simulink library "focLib"  (R2023a)
settings: Solver=VariableStepAuto  StartTime=0.0  StopTime=10.0  RelTol=1e-3
undefined symbols (not defined in the file): availableSpeedModes, ctrl_limits, Down, focp_tune_cur_Ki, focp_tune_cur_Kp, focp_tune_iq_max, focp_tune_iq_min, focp_tune_spd_Ki, focp_tune_spd_Kp, focp_tune_udc_max, GPTRIP1SEL, inverter_DRV8300, PI_params, pmsm_ECI6360, PU_System, target_f2838, Ts, Ts_motor, Ts_simulink, Ts_speed, TZ1, Up
libraries: simulink x31, c2802xlib x12, idelinklib_common x8, mcbcontrolslib x8, c280xlib x7, mcbpositiondecoderlib x7, slpidlib x5, c2837xDlib x2, c2838xlib x1, autolibpmsminterior x1, mcbplantlib x1, autolibpmsmexterior x1
(part 1 of 3)
Description:
  | FOC-Framework Komponentenbibliothek. Aus impmodel erzeugt durch foc_build_library am 2026-11-03 11:16
settings Model: Creator=Student  LastModifiedBy=Student

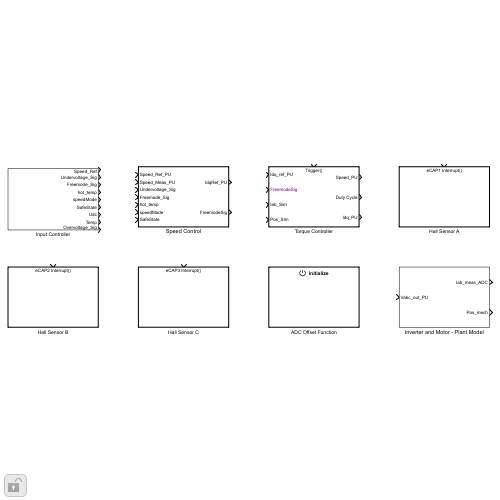
[thumbnail: Simulink's stored preview of the top-level diagram]
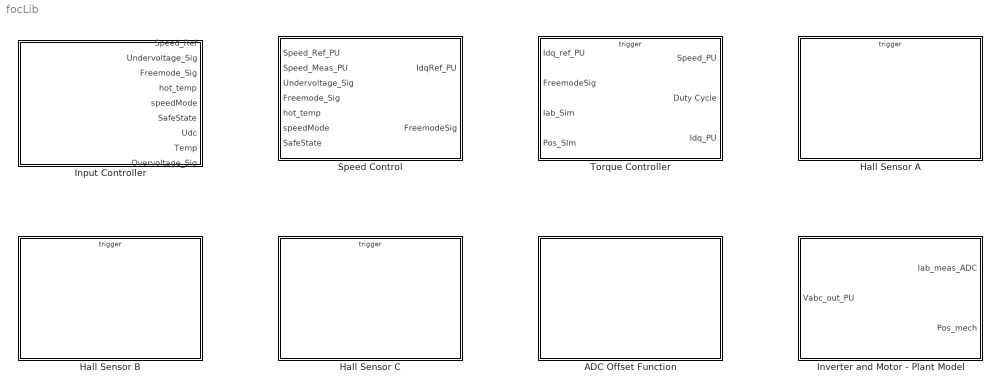
== system focLib ==
  ADC Offset Function : Subsystem  TreatAsAtomicUnit=on
  Hall Sensor A : Subsystem
  Hall Sensor B : Subsystem
  Hall Sensor C : Subsystem
  Input Controller : Subsystem
  Inverter and Motor - Plant Model : Subsystem
  Speed Control : Subsystem  TreatAsAtomicUnit=on  SystemSampleTime=Ts_speed
  Torque Controller : Subsystem

== system focLib/ADC Offset Function ==
  "Calculate ADC Offset " : Subsystem  Priority=1001  TreatAsAtomicUnit=on
  Constant : Constant  Value=inverter_DRV8300.ADCOffsetCalibEnable
  Default ADC Offset : Subsystem  Priority=1001  TreatAsAtomicUnit=on
  Event Listener : EventListener  DisableCoverage=on  EventName=reset
  NOT : Logic  Operator=NOT  IconShape=distinctive  AllPortsSameDT=off  OutDataTypeStr=boolean
  wires:
  NOT/1 -> Default ADC Offset/Enable
  Constant/1 -> "Calculate ADC Offset "/Enable, NOT/1

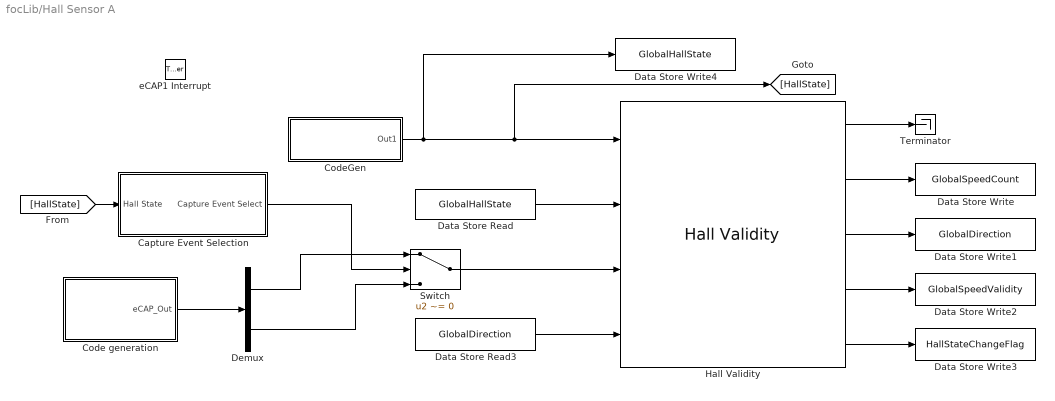
== system focLib/Hall Sensor A ==
  eCAP1 Interrupt : TriggerPort  TriggerType=function-call  VariantControl=(inherit)  PortDimensions=1
  Capture Event Selection : Subsystem
  Code generation : Subsystem
  CodeGen : Subsystem
  Data Store Read : DataStoreRead  DataStoreName=GlobalHallState  IndexOptions=Index vector (dialog)  Indices=1  OutputSizes=1
  Data Store Read3 : DataStoreRead  DataStoreName=GlobalDirection  IndexOptions=Index vector (dialog)  Indices=1  OutputSizes=1
  Data Store Write : DataStoreWrite  DataStoreName=GlobalSpeedCount  IndexOptions=Index vector (dialog)  Indices=1  OutputSizes=1
  Data Store Write1 : DataStoreWrite  DataStoreName=GlobalDirection  IndexOptions=Index vector (dialog)  Indices=1  OutputSizes=1
  Data Store Write2 : DataStoreWrite  DataStoreName=GlobalSpeedValidity  IndexOptions=Index vector (dialog)  Indices=1  OutputSizes=1
  Data Store Write3 : DataStoreWrite  DataStoreName=HallStateChangeFlag  IndexOptions=Index vector (dialog)  Indices=1  OutputSizes=1
  Data Store Write4 : DataStoreWrite  DataStoreName=GlobalHallState  IndexOptions=Index vector (dialog)  Indices=1  OutputSizes=1
  Demux : Demux  Outputs=2
  Hall Validity : mcbpositiondecoderlib/Hall Validity  hallSequence=ABC  sequence=[5,4,6,2,3,1]  CounterSize=32 bits
      settings: LibrarySourceBlock=mcblib/Sensor Decoders/Hall Validity
  Switch : Switch  Criteria=u2 ~= 0  SaturateOnIntegerOverflow=off  InputSameDT=off
  Terminator : Terminator
  wires:
  Demux/2 -> Switch/3
  Demux/1 -> Switch/1
  Data Store Read/1 -> Hall Validity/2
  Code generation/1(eCAP_Out) -> Demux/1
  Capture Event Selection/1(Capture Event Select) -> Switch/2
  Switch/1 -> Hall Validity/3
  [HallState] -> Capture Event Selection/1(Hall State)
  Hall Validity/3 -> Data Store Write1/1
  Hall Validity/2 -> Data Store Write/1
  CodeGen/1(Out1) -> Data Store Write4/1, [HallState], Hall Validity/1
  Data Store Read3/1 -> Hall Validity/4
  Hall Validity/5 -> Data Store Write3/1
  Hall Validity/1 -> Terminator/1
  Hall Validity/4 -> Data Store Write2/1

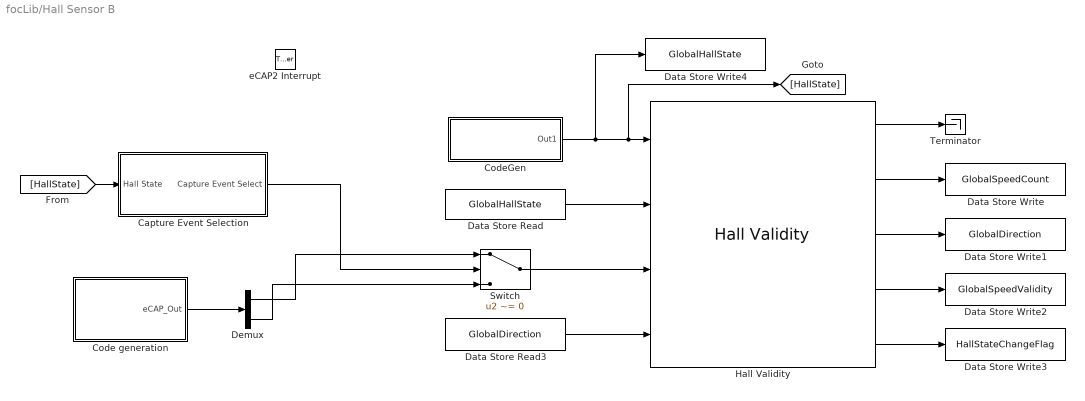
== system focLib/Hall Sensor B ==
  eCAP2 Interrupt : TriggerPort  TriggerType=function-call  VariantControl=(inherit)  PortDimensions=1
  Capture Event Selection : Subsystem
  Code generation : Subsystem
  CodeGen : Subsystem
  Data Store Read : DataStoreRead  DataStoreName=GlobalHallState  IndexOptions=Index vector (dialog)  Indices=1  OutputSizes=1
  Data Store Read3 : DataStoreRead  DataStoreName=GlobalDirection  IndexOptions=Index vector (dialog)  Indices=1  OutputSizes=1
  Data Store Write : DataStoreWrite  DataStoreName=GlobalSpeedCount  IndexOptions=Index vector (dialog)  Indices=1  OutputSizes=1
  Data Store Write1 : DataStoreWrite  DataStoreName=GlobalDirection  IndexOptions=Index vector (dialog)  Indices=1  OutputSizes=1
  Data Store Write2 : DataStoreWrite  DataStoreName=GlobalSpeedValidity  IndexOptions=Index vector (dialog)  Indices=1  OutputSizes=1
  Data Store Write3 : DataStoreWrite  DataStoreName=HallStateChangeFlag  IndexOptions=Index vector (dialog)  Indices=1  OutputSizes=1
  Data Store Write4 : DataStoreWrite  DataStoreName=GlobalHallState  IndexOptions=Index vector (dialog)  Indices=1  OutputSizes=1
  Demux : Demux  Outputs=2
  Hall Validity : mcbpositiondecoderlib/Hall Validity  hallSequence=ABC  sequence=[5,4,6,2,3,1]  CounterSize=32 bits
      settings: LibrarySourceBlock=mcblib/Sensor Decoders/Hall Validity
  Switch : Switch  Criteria=u2 ~= 0  SaturateOnIntegerOverflow=off  InputSameDT=off
  Terminator : Terminator
  wires:
  Data Store Read/1 -> Hall Validity/2
  Switch/1 -> Hall Validity/3
  Demux/2 -> Switch/3
  Demux/1 -> Switch/1
  Code generation/1(eCAP_Out) -> Demux/1
  [HallState] -> Capture Event Selection/1(Hall State)
  Capture Event Selection/1(Capture Event Select) -> Switch/2
  Hall Validity/4 -> Data Store Write2/1
  Hall Validity/1 -> Terminator/1
  Hall Validity/5 -> Data Store Write3/1
  Data Store Read3/1 -> Hall Validity/4
  CodeGen/1(Out1) -> Data Store Write4/1, Hall Validity/1, [HallState]
  Hall Validity/2 -> Data Store Write/1
  Hall Validity/3 -> Data Store Write1/1

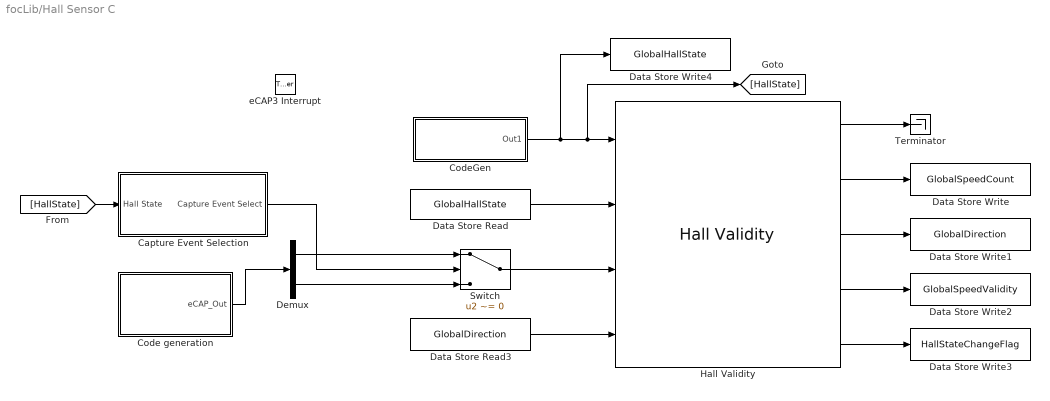
== system focLib/Hall Sensor C ==
  eCAP3 Interrupt : TriggerPort  TriggerType=function-call  VariantControl=(inherit)  PortDimensions=1
  Capture Event Selection : Subsystem
  Code generation : Subsystem
  CodeGen : Subsystem
  Data Store Read : DataStoreRead  DataStoreName=GlobalHallState  IndexOptions=Index vector (dialog)  Indices=1  OutputSizes=1
  Data Store Read3 : DataStoreRead  DataStoreName=GlobalDirection  IndexOptions=Index vector (dialog)  Indices=1  OutputSizes=1
  Data Store Write : DataStoreWrite  DataStoreName=GlobalSpeedCount  IndexOptions=Index vector (dialog)  Indices=1  OutputSizes=1
  Data Store Write1 : DataStoreWrite  DataStoreName=GlobalDirection  IndexOptions=Index vector (dialog)  Indices=1  OutputSizes=1
  Data Store Write2 : DataStoreWrite  DataStoreName=GlobalSpeedValidity  IndexOptions=Index vector (dialog)  Indices=1  OutputSizes=1
  Data Store Write3 : DataStoreWrite  DataStoreName=HallStateChangeFlag  IndexOptions=Index vector (dialog)  Indices=1  OutputSizes=1
  Data Store Write4 : DataStoreWrite  DataStoreName=GlobalHallState  IndexOptions=Index vector (dialog)  Indices=1  OutputSizes=1
  Demux : Demux  Outputs=2
  Hall Validity : mcbpositiondecoderlib/Hall Validity  hallSequence=ABC  sequence=[5,4,6,2,3,1]  CounterSize=32 bits
      settings: LibrarySourceBlock=mcblib/Sensor Decoders/Hall Validity
  Switch : Switch  Criteria=u2 ~= 0  SaturateOnIntegerOverflow=off  InputSameDT=off
  Terminator : Terminator
  wires:
  Data Store Read/1 -> Hall Validity/2
  Capture Event Selection/1(Capture Event Select) -> Switch/2
  Demux/2 -> Switch/3
  Demux/1 -> Switch/1
  Code generation/1(eCAP_Out) -> Demux/1
  Switch/1 -> Hall Validity/3
  [HallState] -> Capture Event Selection/1(Hall State)
  Hall Validity/3 -> Data Store Write1/1
  Hall Validity/2 -> Data Store Write/1
  CodeGen/1(Out1) -> Hall Validity/1, [HallState], Data Store Write4/1
  Data Store Read3/1 -> Hall Validity/4
  Hall Validity/5 -> Data Store Write3/1
  Hall Validity/1 -> Terminator/1
  Hall Validity/4 -> Data Store Write2/1

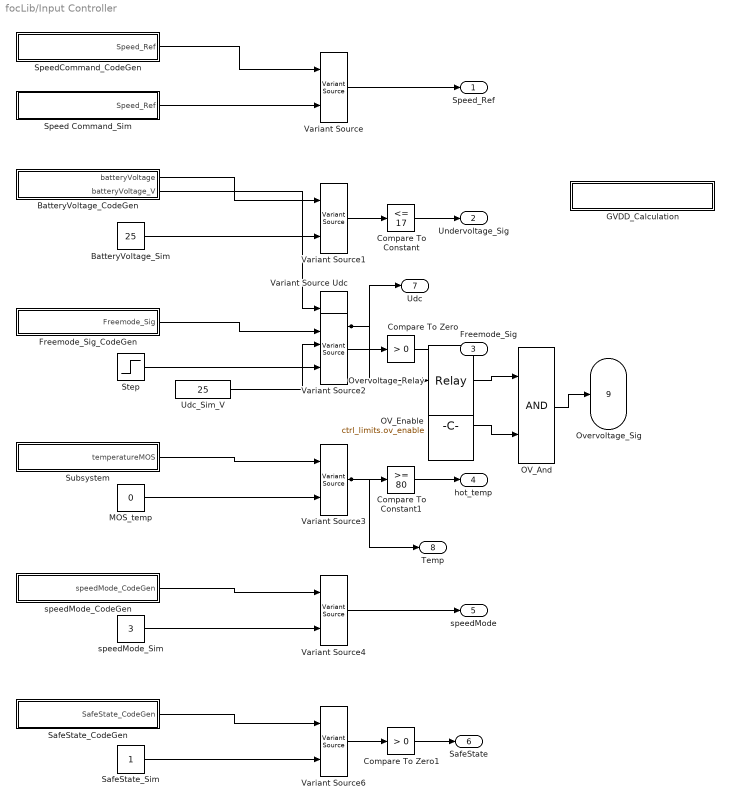
== system focLib/Input Controller ==
  BatteryVoltage_CodeGen : Subsystem
  BatteryVoltage_Sim : Constant  Value=25  OutDataTypeStr=uint16  SampleTime=0.2
  Compare To Constant : simulink/Logic and Bit Operations/Compare To Constant  relop=<=  const=17  OutDataTypeStr=boolean
  Compare To Constant1 : simulink/Logic and Bit Operations/Compare To Constant  relop=>=  const=80  OutDataTypeStr=boolean
  Compare To Zero : simulink/Logic and Bit Operations/Compare To Zero  relop=>  OutDataTypeStr=boolean
  Compare To Zero1 : simulink/Logic and Bit Operations/Compare To Zero  relop=>  OutDataTypeStr=boolean
  Freemode_Sig_CodeGen : Subsystem
  GVDD_Calculation : Subsystem
  MOS_temp : Constant  Value=0  OutDataTypeStr=uint16  SampleTime=0.2
  OV_And : Logic  AllPortsSameDT=off  OutDataTypeStr=boolean
  OV_Enable : Constant  Value=ctrl_limits.ov_enable  OutDataTypeStr=boolean
  Overvoltage_Relay : Relay  OnSwitchValue=focp_tune_udc_max  OffSwitchValue=focp_tune_udc_max - ctrl_limits.Udc_hyst  OutDataTypeStr=boolean
  SafeState_CodeGen : Subsystem
  SafeState_Sim : Constant  OutDataTypeStr=uint8  SampleTime=0.2
  Speed Command_Sim : Subsystem
  SpeedCommand_CodeGen : Subsystem
  Step : Step  Time=10  After=0  SampleTime=0.2
  Subsystem : Subsystem
  Udc_Sim_V : Constant  Value=25  OutDataTypeStr=single
  Variant Source{,1..4,6} (6 alike) : VariantSource  VariantControlMode=sim codegen switching
  Variant Source Udc : VariantSource  VariantControlMode=sim codegen switching
  speedMode_CodeGen : Subsystem
  speedMode_Sim : Constant  Value=3  OutDataTypeStr=uint16  SampleTime=0.2
  Speed_Ref : Outport
  Undervoltage_Sig : Outport  Port=2
  Freemode_Sig : Outport  Port=3
  hot_temp : Outport  Port=4
  speedMode : Outport  Port=5
  SafeState : Outport  Port=6
  Udc : Outport  Port=7
  Temp : Outport  Port=8
  Overvoltage_Sig : Outport  Port=9
  wires:
  Compare To Zero1/1 -> SafeState/1
  SafeState_CodeGen/1(SafeState_CodeGen) -> Variant Source6/1
  SafeState_Sim/1 -> Variant Source6/2
  Variant Source6/1 -> Compare To Zero1/1
  Compare To Zero/1 -> Freemode_Sig/1
  speedMode_CodeGen/1(speedMode_CodeGen) -> Variant Source4/1
  speedMode_Sim/1 -> Variant Source4/2
  Variant Source4/1 -> speedMode/1
  Compare To Constant1/1 -> hot_temp/1
  Variant Source3/1 -> Compare To Constant1/1, Temp/1
  MOS_temp/1 -> Variant Source3/2
  Subsystem/1(temperatureMOS) -> Variant Source3/1
  Freemode_Sig_CodeGen/1(Freemode_Sig) -> Variant Source2/1
  Step/1 -> Variant Source2/2
  Variant Source2/1 -> Compare To Zero/1
  Compare To Constant/1 -> Undervoltage_Sig/1
  BatteryVoltage_Sim/1 -> Variant Source1/2
  BatteryVoltage_CodeGen/1(batteryVoltage) -> Variant Source1/1
  Variant Source1/1 -> Compare To Constant/1
  Speed Command_Sim/1(Speed_Ref) -> Variant Source/2
  SpeedCommand_CodeGen/1(Speed_Ref) -> Variant Source/1
  Variant Source/1 -> Speed_Ref/1
  BatteryVoltage_CodeGen/2(batteryVoltage_V) -> Variant Source Udc/1
  Udc_Sim_V/1 -> Variant Source Udc/2
  Variant Source Udc/1 -> Udc/1, Overvoltage_Relay/1
  Overvoltage_Relay/1 -> OV_And/1
  OV_Enable/1 -> OV_And/2
  OV_And/1 -> Overvoltage_Sig/1

== system focLib/Inverter and Motor - Plant Model ==
  Vabc_out_PU : Inport
  Codegeneration : Subsystem
  Simulation : Subsystem
  Variant Sink : VariantSink  VariantControlMode=sim codegen switching
  Variant Source : VariantSource  VariantControlMode=sim codegen switching
  Variant Source1 : VariantSource  VariantControlMode=sim codegen switching
  Iab_meas_ADC : Outport  VectorParamsAs1DForOutWhenUnconnected=off
  Pos_mech : Outport  Port=2  VectorParamsAs1DForOutWhenUnconnected=off
  wires:
  Vabc_out_PU/1 -> Variant Sink/1
  Simulation/2(Pos_fb_Sim) -> Variant Source1/2
  Variant Sink/2 -> Simulation/1(Duty_Cycles)
  Simulation/1(Iab_fb_Sim) -> Variant Source/2
  Variant Source/1 -> Iab_meas_ADC/1
  Variant Sink/1 -> Codegeneration/1(Duty_Cycles)
  Variant Source1/1 -> Pos_mech/1
  Codegeneration/1(Iab_fb_Sim) -> Variant Source/1
  Codegeneration/2(Pos_fb_Sim) -> Variant Source1/1

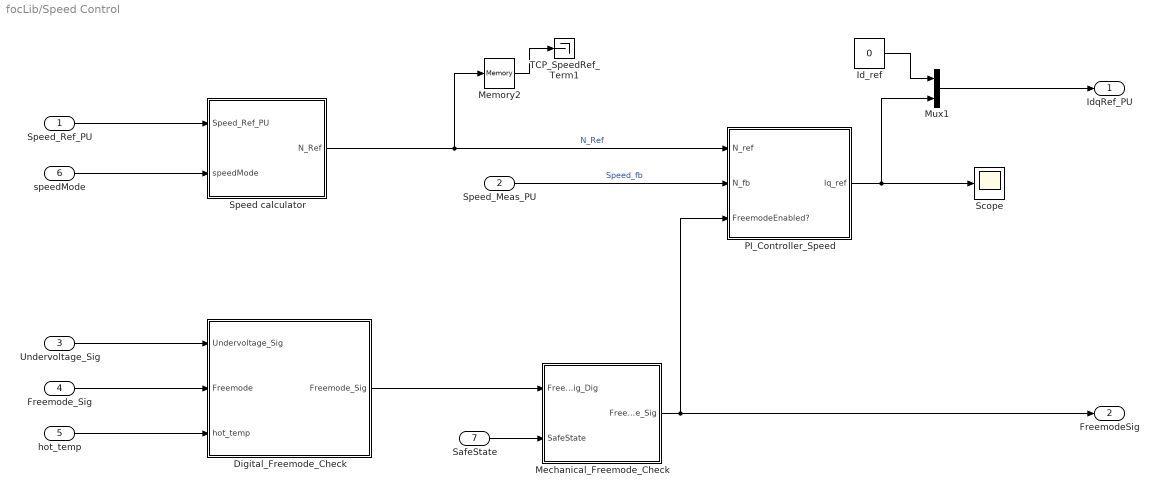
== system focLib/Speed Control ==
  Speed_Ref_PU : Inport
  Speed_Meas_PU : Inport  Port=2
  Undervoltage_Sig : Inport  Port=3
  Freemode_Sig : Inport  Port=4
  hot_temp : Inport  Port=5
  speedMode : Inport  Port=6
  SafeState : Inport  Port=7
  Digital_Freemode_Check : Subsystem  TreatAsAtomicUnit=on
  Id_ref : Constant  Value=0  OutDataTypeStr=fixdt(1,32,17)  SampleTime=Ts_speed
  Mechanical_Freemode_Check : Subsystem
  Memory2 : Memory  InheritSampleTime=on
  Mux1 : Mux  Inputs=2
  PI_Controller_Speed : Subsystem  TreatAsAtomicUnit=on  SystemSampleTime=Ts_speed
  Scope : Scope
  Speed calculator : Subsystem
  TCP_SpeedRef_Term1 : Terminator
  IdqRef_PU : Outport  VectorParamsAs1DForOutWhenUnconnected=off
  FreemodeSig : Outport  Port=2  VectorParamsAs1DForOutWhenUnconnected=off
  wires:
  Mechanical_Freemode_Check/1(Freemode_Sig) -> FreemodeSig/1, PI_Controller_Speed/3("  FreemodeEnabled?")
  Digital_Freemode_Check/1("Freemode_Sig  ") -> Mechanical_Freemode_Check/1(Freemode_Sig_Dig)
  PI_Controller_Speed/1(Iq_ref) -> Mux1/2, Scope/1
  SafeState/1 -> Mechanical_Freemode_Check/2(SafeState)
  Speed_Ref_PU/1 -> Speed calculator/1(Speed_Ref_PU)
  Speed calculator/1(N_Ref) -> PI_Controller_Speed/1(N_ref), Memory2/1  "N_Ref"
  Mux1/1 -> IdqRef_PU/1
  Speed_Meas_PU/1 -> PI_Controller_Speed/2(N_fb)  "Speed_fb"
  hot_temp/1 -> Digital_Freemode_Check/3(hot_temp)
  Undervoltage_Sig/1 -> Digital_Freemode_Check/1(Undervoltage_Sig)
  Freemode_Sig/1 -> Digital_Freemode_Check/2(Freemode)
  speedMode/1 -> Speed calculator/2(speedMode)
  Id_ref/1 -> Mux1/1
  Memory2/1 -> TCP_SpeedRef_Term1/1

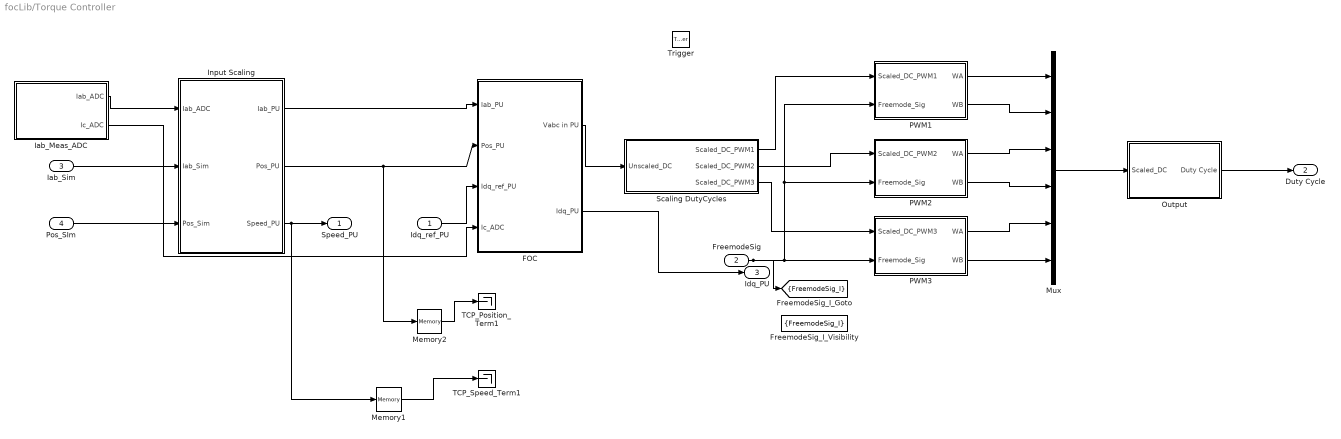
== system focLib/Torque Controller ==
  Idq_ref_PU : Inport
  FreemodeSig : Inport  Port=2
  Iab_Sim : Inport  Port=3
  Pos_SIm : Inport  Port=4
  Trigger : TriggerPort  TriggerType=function-call  VariantControl=(inherit)  PortDimensions=1
  FOC : Subsystem
  FreemodeSig_I_Visibility : GotoTagVisibility  GotoTag=FreemodeSig_I
  Iab_Meas_ADC : Subsystem
  Input Scaling : Subsystem
  Memory1 : Memory  InheritSampleTime=on
  Memory2 : Memory  InheritSampleTime=on
  Mux : Mux  Inputs=6
  Output : Subsystem
  PWM1 : Subsystem
  PWM2 : Subsystem
  PWM3 : Subsystem
  Scaling DutyCycles : Subsystem
  TCP_Position_Term1 : Terminator
  TCP_Speed_Term1 : Terminator
  Speed_PU : Outport
  Duty Cycle : Outport  Port=2
  Idq_PU : Outport  Port=3
  tag scope: FreemodeSig_I=scoped
  wires:
  Input Scaling/2(Pos_PU) -> FOC/2(Pos_PU), Memory2/1
  Input Scaling/1(Iab_PU) -> FOC/1(Iab_PU)
  Mux/1 -> Output/1(Scaled_DC)
  Output/1(Duty Cycle) -> Duty Cycle/1
  FOC/1(Vabc in PU) -> Scaling DutyCycles/1(Unscaled_DC)
  FreemodeSig/1 -> PWM2/2(Freemode_Sig), PWM1/2(Freemode_Sig), PWM3/2(Freemode_Sig), [FreemodeSig_I]
  PWM3/1(WA) -> Mux/5
  PWM2/2(WB) -> Mux/4
  Scaling DutyCycles/1(Scaled_DC_PWM1) -> PWM1/1(Scaled_DC_PWM1)
  PWM1/1(WA) -> Mux/1
  Scaling DutyCycles/3(Scaled_DC_PWM3) -> PWM3/1(Scaled_DC_PWM3)
  PWM2/1(WA) -> Mux/3
  Scaling DutyCycles/2(Scaled_DC_PWM2) -> PWM2/1(Scaled_DC_PWM2)
  PWM3/2(WB) -> Mux/6
  PWM1/2(WB) -> Mux/2
  Pos_SIm/1 -> Input Scaling/3(Pos_Sim)
  Iab_Sim/1 -> Input Scaling/2(Iab_Sim)
  Iab_Meas_ADC/1(Iab_ADC) -> Input Scaling/1(Iab_ADC)
  Idq_ref_PU/1 -> FOC/3(Idq_ref_PU)
  Input Scaling/3(Speed_PU) -> Speed_PU/1, Memory1/1
  FOC/2(Idq_PU) -> Idq_PU/1
  Memory2/1 -> TCP_Position_Term1/1
  Memory1/1 -> TCP_Speed_Term1/1
  Iab_Meas_ADC/2(Ic_ADC) -> FOC/4(Ic_ADC)

== system focLib/ADC Offset Function/Calculate ADC Offset  ==
  Enable : EnablePort
  Constant : Constant  Value=8
  Constant1 : Constant  Value=inverter_DRV8300.CtSensOffsetMax  OutDataTypeStr=Inherit: Inherit via back propagation
  Constant2 : Constant  Value=inverter_DRV8300.CtSensOffsetMin  OutDataTypeStr=Inherit: Inherit via back propagation
  Divide : Product  Inputs=*/  OutDataTypeStr=uint16
  Divide1 : Product  Inputs=*/  OutDataTypeStr=uint16
  For Iterator Subsystem : Subsystem  TreatAsAtomicUnit=on
  If : If  NumInputs=3  IfExpression=u1 > u3 & u1 < u2
  If Action Subsystem : Subsystem  TreatAsAtomicUnit=on
  If Action Subsystem1 : Subsystem  TreatAsAtomicUnit=on
  If Action Subsystem2 : Subsystem  TreatAsAtomicUnit=on
  If Action Subsystem3 : Subsystem  TreatAsAtomicUnit=on
  If1 : If  NumInputs=3  IfExpression=u1 > u3 & u1 < u2
  wires:
  Divide/1 -> If/1, If Action Subsystem/1(In1)
  Constant/1 -> Divide1/2, Divide/2
  Divide1/1 -> If Action Subsystem2/1(In1), If1/1
  Constant1/1 -> If1/2, If/2
  Constant2/1 -> If1/3, If/3
  If/1 -> If Action Subsystem/Action
  For Iterator Subsystem/2(Out2) -> Divide1/1
  If/2 -> If Action Subsystem1/Action
  If1/1 -> If Action Subsystem2/Action
  If1/2 -> If Action Subsystem3/Action
  For Iterator Subsystem/1(Out1) -> Divide/1

== system focLib/ADC Offset Function/Default ADC Offset ==
  Enable : EnablePort
  Constant : Constant  Value=inverter_DRV8300.CtSensAOffset  OutDataTypeStr=Inherit: Inherit via back propagation
  Constant1 : Constant  Value=inverter_DRV8300.CtSensBOffset  OutDataTypeStr=Inherit: Inherit via back propagation
  Data Store Write1 : DataStoreWrite  DataStoreName=IaOffset  IndexOptions=Index vector (dialog)  Indices=1  OutputSizes=1
  Data Store Write2 : DataStoreWrite  DataStoreName=IbOffset  IndexOptions=Index vector (dialog)  Indices=1  OutputSizes=1
  wires:
  Constant1/1 -> Data Store Write2/1
  Constant/1 -> Data Store Write1/1

== system focLib/Hall Sensor A/Capture Event Selection ==
  Hall State : Inport
  If : If  IfExpression=(u1 == 5 | u1 == 3)
  Merge : Merge
  Output 0 : Subsystem  TreatAsAtomicUnit=on
  Output 1 : Subsystem  TreatAsAtomicUnit=on
  Capture Event Select : Outport
  wires:
  Output 1/1(Out1) -> Merge/1
  If/1 -> Output 1/Action
  If/2 -> Output 0/Action
  Output 0/1(Out1) -> Merge/2
  Merge/1 -> Capture Event Select/1
  Hall State/1 -> If/1

== system focLib/Hall Sensor A/Code generation ==
  eCAP : c280xlib/eCAP  operatingMode=eCAP  selectCAPx=eCAP1  offsetValue=0  counterSynIn=off  enableCounter=off  syncOutput=Pass through  sampleTime=-1  eventPrescaler=0  selectMode=Continuous  enableOneShot=off  stopValue=Capture Event 2  resetEv1Ts=on  ev1Polarity=Rising Edge  resetEv2Ts=on  ev2Polarity=Falling Edge  resetEv3Ts=off  ev3Polarity=Rising Edge  resetEv4Ts=off  ev4Polarity=Rising Edge  tSCntrDataType=uint32  capEvFlag=off  capFlagDataType=uint32  overFlowFlag=off  overFlowFlagDataType=uint16  periodUnit=Seconds  periodSource=Specify via dialog  waveformPeriod=0.001  dutyUnit=Percentages  dutySource=Specify via dialog  dutyCycle=50  outputPolarity=Active High  enableCEVT1Int=on  enableCEVT2Int=on  enableCEVT3Int=off  enableCEVT4Int=off  enableCTROVFInt=on  enablePRDInt=off  enableCMPInt=off
      settings: LibrarySourceBlock=c2838xlib/eCAP
  eCAP_Out : Outport
  wires:
  eCAP/1 -> eCAP_Out/1

== system focLib/Hall Sensor A/CodeGen ==
  Bitwise OR : simulink/Logic and Bit Operations/Bitwise Operator  logicop=OR  UseBitMask=off  NumInputPorts=3  BitMask=bin2dec('11011001')  BitMaskRealWorld=Stored Integer
      settings: LibrarySourceBlock=|
      | simulink/Quick Insert/Logic and Bit
      | Operations/Bitwise OR
  Data Store Write : DataStoreWrite  DataStoreName=HallC  IndexOptions=Index vector (dialog)  Indices=1  OutputSizes=1
  Data Store Write1 : DataStoreWrite  DataStoreName=HallB  IndexOptions=Index vector (dialog)  Indices=1  OutputSizes=1
  Data Store Write2 : DataStoreWrite  DataStoreName=HallA  IndexOptions=Index vector (dialog)  Indices=1  OutputSizes=1
  Data Type Conversion : DataTypeConversion  OutDataTypeStr=uint32  ConvertRealWorld=Stored Integer (SI)  SaturateOnIntegerOverflow=off  RndMeth=Floor
  GPIO 24 Hall_A : simulink/Logic and Bit Operations/Bitwise Operator  logicop=AND  UseBitMask=on  BitMask=hex2dec('1000000')  BitMaskRealWorld=Stored Integer
      settings: LibrarySourceBlock=|
      | simulink/Quick Insert/Logic and Bit
      | Operations/Bitwise AND
  GPIO 25 Hall_B : simulink/Logic and Bit Operations/Bitwise Operator  logicop=AND  UseBitMask=on  BitMask=hex2dec('2000000')  BitMaskRealWorld=Stored Integer
      settings: LibrarySourceBlock=|
      | simulink/Quick Insert/Logic and Bit
      | Operations/Bitwise AND
  GPIO 26 Hall_C : simulink/Logic and Bit Operations/Bitwise Operator  logicop=AND  UseBitMask=on  BitMask=hex2dec('4000000')  BitMaskRealWorld=Stored Integer
      settings: LibrarySourceBlock=|
      | simulink/Quick Insert/Logic and Bit
      | Operations/Bitwise AND
  Memory Copy : idelinklib_common/Memory Copy  copyFrom=Specified source code symbol  copyFromAddressSource=Specify via dialog  copyFromAddress=hex2dec('00001000')  copyFromSrcCode=&GpioDataRegs.GPADAT.all  dataTypeFrom=uint32  dataDimensionFrom=1  useOffsetFrom=off  offsetFromSrc=Specify via dialog  offsetFrom=0  strideFrom=1  copyTo=Output port  copyToAddressSource=Specify via dialog  copyToAddress=hex2dec('00002000')  copyToSrcCode=myVariableDst  dataTypeTo=uint32  useOffsetTo=off  offsetToSrc=Specify via dialog  offsetTo=0  strideTo=1  sampleTime=-1  useInitValue=off  initValueSrc=Specify constant value  initValue=1  initValueSrcCode=myInitValueVariable  useAsMask=off  maskOperator=bitwise AND  useTermValue=off  termValue=1  isRealtimeEnabled=off  emitCCBeforeWrite=off  CCBeforeWrite=/* Custom Code Before Write*/  emitCCAfterWrite=off  CCAfterWrite=/* Custom Code After Write*/
  Shift Arithmetic : ArithShift  BitShiftNumber=26
  Shift Arithmetic1 : ArithShift  BitShiftNumber=24
  Shift Arithmetic2 : ArithShift  BitShiftNumber=22
  Out1 : Outport
  wires:
  GPIO 25 Hall_B/1 -> Shift Arithmetic1/1
  Memory Copy/1 -> GPIO 26 Hall_C/1, GPIO 24 Hall_A/1, GPIO 25 Hall_B/1
  Shift Arithmetic2/1 -> Bitwise OR/3, Data Store Write2/1
  Shift Arithmetic1/1 -> Bitwise OR/2, Data Store Write1/1
  GPIO 24 Hall_A/1 -> Shift Arithmetic2/1
  Shift Arithmetic/1 -> Bitwise OR/1, Data Store Write/1
  Bitwise OR/1 -> Data Type Conversion/1
  GPIO 26 Hall_C/1 -> Shift Arithmetic/1
  Data Type Conversion/1 -> Out1/1

== system focLib/Hall Sensor B/Capture Event Selection ==
  Hall State : Inport
  If : If  IfExpression=(u1 == 3 | u1 == 6)
  Merge : Merge
  Output 0 : Subsystem  TreatAsAtomicUnit=on
  Output 1 : Subsystem  TreatAsAtomicUnit=on
  Capture Event Select : Outport
  wires:
  Output 1/1(Out1) -> Merge/1
  If/1 -> Output 1/Action
  If/2 -> Output 0/Action
  Output 0/1(Out1) -> Merge/2
  Merge/1 -> Capture Event Select/1
  Hall State/1 -> If/1

== system focLib/Hall Sensor B/Code generation ==
  eCAP : c280xlib/eCAP  operatingMode=eCAP  selectCAPx=eCAP2  offsetValue=0  counterSynIn=off  enableCounter=off  syncOutput=Pass through  sampleTime=-1  eventPrescaler=0  selectMode=Continuous  enableOneShot=off  stopValue=Capture Event 2  resetEv1Ts=on  ev1Polarity=Rising Edge  resetEv2Ts=on  ev2Polarity=Falling Edge  resetEv3Ts=off  ev3Polarity=Rising Edge  resetEv4Ts=off  ev4Polarity=Rising Edge  tSCntrDataType=uint32  capEvFlag=off  capFlagDataType=uint16  overFlowFlag=off  overFlowFlagDataType=uint16  periodUnit=Seconds  periodSource=Specify via dialog  waveformPeriod=0.001  dutyUnit=Percentages  dutySource=Specify via dialog  dutyCycle=50  outputPolarity=Active High  enableCEVT1Int=on  enableCEVT2Int=on  enableCEVT3Int=off  enableCEVT4Int=off  enableCTROVFInt=on  enablePRDInt=off  enableCMPInt=off
      settings: LibrarySourceBlock=c2838xlib/eCAP
  eCAP_Out : Outport
  wires:
  eCAP/1 -> eCAP_Out/1

== system focLib/Hall Sensor B/CodeGen ==
  Bitwise OR : simulink/Logic and Bit Operations/Bitwise Operator  logicop=OR  UseBitMask=off  NumInputPorts=3  BitMask=bin2dec('11011001')  BitMaskRealWorld=Stored Integer
      settings: LibrarySourceBlock=|
      | simulink/Quick Insert/Logic and Bit
      | Operations/Bitwise OR
  Data Store Write : DataStoreWrite  DataStoreName=HallC  IndexOptions=Index vector (dialog)  Indices=1  OutputSizes=1
  Data Store Write1 : DataStoreWrite  DataStoreName=HallB  IndexOptions=Index vector (dialog)  Indices=1  OutputSizes=1
  Data Store Write2 : DataStoreWrite  DataStoreName=HallA  IndexOptions=Index vector (dialog)  Indices=1  OutputSizes=1
  Data Type Conversion : DataTypeConversion  OutDataTypeStr=uint32  ConvertRealWorld=Stored Integer (SI)  SaturateOnIntegerOverflow=off  RndMeth=Floor
  GPIO 24 Hall_A : simulink/Logic and Bit Operations/Bitwise Operator  logicop=AND  UseBitMask=on  BitMask=hex2dec('1000000')  BitMaskRealWorld=Stored Integer
      settings: LibrarySourceBlock=|
      | simulink/Quick Insert/Logic and Bit
      | Operations/Bitwise AND
  GPIO 25 Hall_B : simulink/Logic and Bit Operations/Bitwise Operator  logicop=AND  UseBitMask=on  BitMask=hex2dec('2000000')  BitMaskRealWorld=Stored Integer
      settings: LibrarySourceBlock=|
      | simulink/Quick Insert/Logic and Bit
      | Operations/Bitwise AND
  GPIO 26 Hall_C : simulink/Logic and Bit Operations/Bitwise Operator  logicop=AND  UseBitMask=on  BitMask=hex2dec('4000000')  BitMaskRealWorld=Stored Integer
      settings: LibrarySourceBlock=|
      | simulink/Quick Insert/Logic and Bit
      | Operations/Bitwise AND
  Memory Copy : idelinklib_common/Memory Copy  copyFrom=Specified source code symbol  copyFromAddressSource=Specify via dialog  copyFromAddress=hex2dec('00001000')  copyFromSrcCode=&GpioDataRegs.GPADAT.all  dataTypeFrom=uint32  dataDimensionFrom=1  useOffsetFrom=off  offsetFromSrc=Specify via dialog  offsetFrom=0  strideFrom=1  copyTo=Output port  copyToAddressSource=Specify via dialog  copyToAddress=hex2dec('00002000')  copyToSrcCode=myVariableDst  dataTypeTo=uint32  useOffsetTo=off  offsetToSrc=Specify via dialog  offsetTo=0  strideTo=1  sampleTime=-1  useInitValue=off  initValueSrc=Specify constant value  initValue=1  initValueSrcCode=myInitValueVariable  useAsMask=off  maskOperator=bitwise AND  useTermValue=off  termValue=1  isRealtimeEnabled=off  emitCCBeforeWrite=off  CCBeforeWrite=/* Custom Code Before Write*/  emitCCAfterWrite=off  CCAfterWrite=/* Custom Code After Write*/
  Shift Arithmetic : ArithShift  BitShiftNumber=26
  Shift Arithmetic1 : ArithShift  BitShiftNumber=24
  Shift Arithmetic2 : ArithShift  BitShiftNumber=22
  Out1 : Outport
  wires:
  GPIO 26 Hall_C/1 -> Shift Arithmetic/1
  GPIO 25 Hall_B/1 -> Shift Arithmetic1/1
  GPIO 24 Hall_A/1 -> Shift Arithmetic2/1
  Bitwise OR/1 -> Data Type Conversion/1
  Shift Arithmetic/1 -> Bitwise OR/1, Data Store Write/1
  Memory Copy/1 -> GPIO 24 Hall_A/1, GPIO 25 Hall_B/1, GPIO 26 Hall_C/1
  Shift Arithmetic1/1 -> Bitwise OR/2, Data Store Write1/1
  Shift Arithmetic2/1 -> Bitwise OR/3, Data Store Write2/1
  Data Type Conversion/1 -> Out1/1

== system focLib/Hall Sensor C/Capture Event Selection ==
  Hall State : Inport
  If : If  IfExpression=(u1 == 5 | u1 == 6)
  Merge : Merge
  Output 0 : Subsystem  TreatAsAtomicUnit=on
  Output 1 : Subsystem  TreatAsAtomicUnit=on
  Capture Event Select : Outport
  wires:
  Output 1/1(Out1) -> Merge/1
  If/1 -> Output 1/Action
  If/2 -> Output 0/Action
  Output 0/1(Out1) -> Merge/2
  Merge/1 -> Capture Event Select/1
  Hall State/1 -> If/1

== system focLib/Hall Sensor C/Code generation ==
  eCAP : c280xlib/eCAP  operatingMode=eCAP  selectCAPx=eCAP3  offsetValue=0  counterSynIn=off  enableCounter=off  syncOutput=Disabled  sampleTime=-1  eventPrescaler=0  selectMode=Continuous  enableOneShot=off  stopValue=Capture Event 2  resetEv1Ts=on  ev1Polarity=Rising Edge  resetEv2Ts=on  ev2Polarity=Falling Edge  resetEv3Ts=off  ev3Polarity=Rising Edge  resetEv4Ts=off  ev4Polarity=Rising Edge  tSCntrDataType=uint32  capEvFlag=off  capFlagDataType=uint16  overFlowFlag=off  overFlowFlagDataType=uint16  periodUnit=Seconds  periodSource=Specify via dialog  waveformPeriod=0.001  dutyUnit=Percentages  dutySource=Specify via dialog  dutyCycle=50  outputPolarity=Active High  enableCEVT1Int=on  enableCEVT2Int=on  enableCEVT3Int=off  enableCEVT4Int=off  enableCTROVFInt=on  enablePRDInt=off  enableCMPInt=off
      settings: LibrarySourceBlock=c2838xlib/eCAP
  eCAP_Out : Outport
  wires:
  eCAP/1 -> eCAP_Out/1

== system focLib/Hall Sensor C/CodeGen ==
  Bitwise OR : simulink/Logic and Bit Operations/Bitwise Operator  logicop=OR  UseBitMask=off  NumInputPorts=3  BitMask=bin2dec('11011001')  BitMaskRealWorld=Stored Integer
      settings: LibrarySourceBlock=|
      | simulink/Quick Insert/Logic and Bit
      | Operations/Bitwise OR
  Data Store Write : DataStoreWrite  DataStoreName=HallC  IndexOptions=Index vector (dialog)  Indices=1  OutputSizes=1
  Data Store Write1 : DataStoreWrite  DataStoreName=HallB  IndexOptions=Index vector (dialog)  Indices=1  OutputSizes=1
  Data Store Write2 : DataStoreWrite  DataStoreName=HallA  IndexOptions=Index vector (dialog)  Indices=1  OutputSizes=1
  Data Type Conversion : DataTypeConversion  OutDataTypeStr=uint32  ConvertRealWorld=Stored Integer (SI)  SaturateOnIntegerOverflow=off  RndMeth=Floor
  GPIO 24 Hall_A : simulink/Logic and Bit Operations/Bitwise Operator  logicop=AND  UseBitMask=on  BitMask=hex2dec('1000000')  BitMaskRealWorld=Stored Integer
      settings: LibrarySourceBlock=|
      | simulink/Quick Insert/Logic and Bit
      | Operations/Bitwise AND
  GPIO 25 Hall_B : simulink/Logic and Bit Operations/Bitwise Operator  logicop=AND  UseBitMask=on  BitMask=hex2dec('2000000')  BitMaskRealWorld=Stored Integer
      settings: LibrarySourceBlock=|
      | simulink/Quick Insert/Logic and Bit
      | Operations/Bitwise AND
  GPIO 26 Hall_C : simulink/Logic and Bit Operations/Bitwise Operator  logicop=AND  UseBitMask=on  BitMask=hex2dec('4000000')  BitMaskRealWorld=Stored Integer
      settings: LibrarySourceBlock=|
      | simulink/Quick Insert/Logic and Bit
      | Operations/Bitwise AND
  Memory Copy : idelinklib_common/Memory Copy  copyFrom=Specified source code symbol  copyFromAddressSource=Specify via dialog  copyFromAddress=hex2dec('00001000')  copyFromSrcCode=&GpioDataRegs.GPADAT.all  dataTypeFrom=uint32  dataDimensionFrom=1  useOffsetFrom=off  offsetFromSrc=Specify via dialog  offsetFrom=0  strideFrom=1  copyTo=Output port  copyToAddressSource=Specify via dialog  copyToAddress=hex2dec('00002000')  copyToSrcCode=myVariableDst  dataTypeTo=uint32  useOffsetTo=off  offsetToSrc=Specify via dialog  offsetTo=0  strideTo=1  sampleTime=-1  useInitValue=off  initValueSrc=Specify constant value  initValue=1  initValueSrcCode=myInitValueVariable  useAsMask=off  maskOperator=bitwise AND  useTermValue=off  termValue=1  isRealtimeEnabled=off  emitCCBeforeWrite=off  CCBeforeWrite=/* Custom Code Before Write*/  emitCCAfterWrite=off  CCAfterWrite=/* Custom Code After Write*/
  Shift Arithmetic : ArithShift  BitShiftNumber=26
  Shift Arithmetic1 : ArithShift  BitShiftNumber=24
  Shift Arithmetic2 : ArithShift  BitShiftNumber=22
  Out1 : Outport
  wires:
  GPIO 26 Hall_C/1 -> Shift Arithmetic/1
  GPIO 25 Hall_B/1 -> Shift Arithmetic1/1
  GPIO 24 Hall_A/1 -> Shift Arithmetic2/1
  Bitwise OR/1 -> Data Type Conversion/1
  Shift Arithmetic/1 -> Bitwise OR/1, Data Store Write/1
  Memory Copy/1 -> GPIO 24 Hall_A/1, GPIO 25 Hall_B/1, GPIO 26 Hall_C/1
  Shift Arithmetic1/1 -> Bitwise OR/2, Data Store Write1/1
  Shift Arithmetic2/1 -> Bitwise OR/3, Data Store Write2/1
  Data Type Conversion/1 -> Out1/1

== system focLib/Input Controller/BatteryVoltage_CodeGen ==
  " " : c2802xlib/ADC  blkParamProc=C2000_Type4  ADCModule=A  samplingMode=Single sample mode  ADCResolution=12-bit (Single-ended input)  useSOC1=SOC3  useSOC2=SOC0_SOC1  SOCAcquisitionWindow=200  SOCTriggerSource=Software  SOCInterruptTrigger=No ADCINT  Ts=0.2  dType=uint16  postInterrupt=off  interruptSel=ADCINT1  ADCINTContinuous=on  endma=off  chdma=1  conv1=ADCINA0  conv2=ADCINA0 and ADCINB0  conv1_Type4=ADCIN5  conv2_Type4=ADCIN0 and ADCIN1
      settings: LibrarySourceBlock=c2838xlib/ADC
  Data Type Conversion : DataTypeConversion  OutDataTypeStr=single  SaturateOnIntegerOverflow=off  RndMeth=Floor
  Data Type Conversion1 : DataTypeConversion  OutDataTypeStr=uint16  RndMeth=Nearest  SaturateOnIntegerOverflow=off
  Divide : Product  Inputs=*/  OutDataTypeStr=Inherit: Same as first input
  Product : Product  OutDataTypeStr=Inherit: Same as first input
  Product2 : Product  OutDataTypeStr=Inherit: Same as first input
  R1+R2 : Constant  Value=100610  OutDataTypeStr=single  SampleTime=-1
  R2 : Constant  Value=3010  OutDataTypeStr=single  SampleTime=-1
  Scaling : Constant  Value=target_f2838.ADC_Vref/target_f2838.ADC_MaxCount  OutDataTypeStr=single  SampleTime=-1
  eCAN Transmit : c280xlib/eCAN Transmit  chipFamily=C280x  useModule=eCAN_A  mailboxNo=1  messageID=hex2dec('110')  messageType=Standard (11-bit identifier)  enableBlockingMode=off  postInterrupt=off  interruptLine=0
      settings: LibrarySourceBlock=c28004xlib/eCAN Transmit
  batteryVoltage : Outport
  batteryVoltage_V : Outport  Port=2
  wires:
  " "/1 -> Data Type Conversion/1
  Data Type Conversion1/1 -> eCAN Transmit/1, batteryVoltage/1
  Product2/1 -> Data Type Conversion1/1, batteryVoltage_V/1
  R1+R2/1 -> Product2/2
  Divide/1 -> Product2/1
  R2/1 -> Divide/2
  Scaling/1 -> Product/2
  Product/1 -> Divide/1
  Data Type Conversion/1 -> Product/1

== system focLib/Input Controller/Freemode_Sig_CodeGen ==
  Data Type Conversion : DataTypeConversion  OutDataTypeStr=fixdt(1,32,17)  SaturateOnIntegerOverflow=off  RndMeth=Floor
  Saturation : Saturate  UpperLimit=1  LowerLimit=0
  Select first element : Selector  InputPortWidth=4  IndexOptions=Index vector (dialog)  Indices=[1]  OutputSizes=1
  Terminator : Terminator
  eCAN Receive : c280xlib/eCAN Receive  chipFamily=C280x  useModule=eCAN_A  mailboxNo=9  messageID=hex2dec('101')  messageType=Standard (11-bit identifier)  enableAcceptanceFiltering=off  messageIDMask=0  sampleTime=0.2  dataType=uint16  outputAction=Output last received values  initValue=0  outputMessageID=off  outputMessageLength=off  outputMessageTimeStamp=off  postInterrupt=off  interruptLine=0
      settings: LibrarySourceBlock=c28004xlib/eCAN Receive
  Freemode_Sig : Outport
  wires:
  Saturation/1 -> Freemode_Sig/1
  Select first element/1 -> Data Type Conversion/1
  Data Type Conversion/1 -> Saturation/1
  eCAN Receive/2 -> Select first element/1
  eCAN Receive/1 -> Terminator/1

== system focLib/Input Controller/GVDD_Calculation ==
  ADC : c2802xlib/ADC  blkParamProc=C2000_Type5  ADCModule=C  samplingMode=Single sample mode  ADCResolution=12-bit (Single-ended input)  useSOC1=SOC4  useSOC2=SOC0_SOC1  SOCAcquisitionWindow=200  SOCTriggerSource=Software  SOCInterruptTrigger=No ADCINT  Ts=0.2  dType=uint16  postInterrupt=off  interruptSel=ADCINT1  ADCINTContinuous=on  endma=off  chdma=1  conv1=ADCINA0  conv2=ADCINA0 and ADCINB0  conv1_Type4=ADCIN3  conv2_Type4=ADCIN0 and ADCIN1
      settings: LibrarySourceBlock=c28004xlib/ADC
  Data Type Conversion : DataTypeConversion  OutDataTypeStr=single  SaturateOnIntegerOverflow=off  RndMeth=Floor
  Data Type Conversion1 : DataTypeConversion  OutDataTypeStr=uint16  RndMeth=Nearest  SaturateOnIntegerOverflow=off
  Divide : Product  Inputs=*/  OutDataTypeStr=Inherit: Same as first input
  Product : Product  OutDataTypeStr=Inherit: Same as first input
  Product2 : Product  OutDataTypeStr=Inherit: Same as first input
  R1+R2 : Constant  Value=100610  OutDataTypeStr=single  SampleTime=-1
  R2 : Constant  Value=3010  OutDataTypeStr=single  SampleTime=-1
  Scaling : Constant  Value=target_f2838.ADC_Vref/target_f2838.ADC_MaxCount  OutDataTypeStr=single  SampleTime=-1
  eCAN Transmit : c280xlib/eCAN Transmit  chipFamily=C280x  useModule=eCAN_A  mailboxNo=2  messageID=hex2dec('111')  messageType=Standard (11-bit identifier)  enableBlockingMode=off  postInterrupt=off  interruptLine=0
      settings: LibrarySourceBlock=c28004xlib/eCAN Transmit
  wires:
  ADC/1 -> Data Type Conversion/1
  Data Type Conversion/1 -> Product/1
  Product/1 -> Divide/1
  Scaling/1 -> Product/2
  R2/1 -> Divide/2
  Divide/1 -> Product2/1
  R1+R2/1 -> Product2/2
  Product2/1 -> Data Type Conversion1/1
  Data Type Conversion1/1 -> eCAN Transmit/1

== system focLib/Input Controller/SafeState_CodeGen ==
  SafeState_Pin : c2838xlib/Digital Input  GPIO_Number=GPIO24~GPIO31  GPIO_Bit0=off  GPIO_Bit1=off  GPIO_Bit2=off  GPIO_Bit3=off  GPIO_Bit4=off  GPIO_Bit5=off  GPIO_Bit6=on  GPIO_Bit7=off  sampleTime=0.2  dataType=boolean  GPIO_Bit0_Qualification=Sync to SYSCLKOUT  GPIO_Bit1_Qualification=Sync to SYSCLKOUT  GPIO_Bit2_Qualification=Sync to SYSCLKOUT  GPIO_Bit3_Qualification=Sync to SYSCLKOUT  GPIO_Bit4_Qualification=Sync to SYSCLKOUT  GPIO_Bit5_Qualification=Sync to SYSCLKOUT  GPIO_Bit6_Qualification=Sync to SYSCLKOUT  GPIO_Bit7_Qualification=Sync to SYSCLKOUT  Qualification_Period=-1
  SafeState_CodeGen : Outport
  wires:
  SafeState_Pin/1 -> SafeState_CodeGen/1

== system focLib/Input Controller/Speed Command_Sim ==
  Data Type Conversion : DataTypeConversion  OutDataTypeStr=fixdt(1,32,17)  SaturateOnIntegerOverflow=off  RndMeth=Floor
  Reversal : Step  Commented=on  Time=5  SampleTime=0.01
  Sine Wave : Sin  Commented=on  Amplitude=0.9  Frequency=0.2  SampleTime=0.01
  Speed_Ref_Final (rpm) : Constant  Commented=on  Value=0  OutDataTypeStr=double  SampleTime=0.01
  Step : Step  After=0.25  SampleTime=0.01
  Switch : Switch  Commented=on  Criteria=u2 > Threshold  SaturateOnIntegerOverflow=off  InputSameDT=off
  Speed_Ref : Outport
  wires:
  Step/1 -> Data Type Conversion/1
  Data Type Conversion/1 -> Speed_Ref/1
  Speed_Ref_Final (rpm)/1 -> Switch/1
  Sine Wave/1 -> Switch/3
  Reversal/1 -> Switch/2

== system focLib/Input Controller/SpeedCommand_CodeGen ==
  note: This Subsystem is essential due to the fact that the voltage at the potentiometer will not reach 3.3 V.
      | At an ADC value bigger than 4000 the output will jump to 4095 (full speed)
  ADC1 : c2802xlib/ADC  blkParamProc=C2000_Type4  ADCModule=A  samplingMode=Single sample mode  ADCResolution=12-bit (Single-ended input)  useSOC1=SOC2  useSOC2=SOC0_SOC1  SOCAcquisitionWindow=200  SOCTriggerSource=Software  SOCInterruptTrigger=No ADCINT  Ts=0.01  dType=uint16  postInterrupt=off  interruptSel=ADCINT1  ADCINTContinuous=on  endma=off  chdma=1  conv1=ADCINA0  conv2=ADCINA0 and ADCINB0  conv1_Type4=ADCIN0  conv2_Type4=ADCIN0 and ADCIN1
      settings: LibrarySourceBlock=c2838xlib/ADC
  Check for SpeedRef : Subsystem
  normalizeADCValue : Gain  Gain=1/4095  OutDataTypeStr=fixdt(1,32,17)  RndMeth=Ceiling
  Speed_Ref : Outport
  wires:
  ADC1/1 -> Check for SpeedRef/1(In1)
  Check for SpeedRef/1(Out1) -> normalizeADCValue/1
  normalizeADCValue/1 -> Speed_Ref/1

== system focLib/Input Controller/Subsystem ==
  ADC1 : c2802xlib/ADC  blkParamProc=C2000_Type4  ADCModule=C  samplingMode=Single sample mode  ADCResolution=12-bit (Single-ended input)  useSOC1=SOC5  useSOC2=SOC0_SOC1  SOCAcquisitionWindow=200  SOCTriggerSource=Software  SOCInterruptTrigger=No ADCINT  Ts=0.2  dType=uint16  postInterrupt=off  interruptSel=ADCINT1  ADCINTContinuous=on  endma=off  chdma=1  conv1=ADCINA0  conv2=ADCINA0 and ADCINB0  conv1_Type4=ADCIN2  conv2_Type4=ADCIN0 and ADCIN1
      settings: LibrarySourceBlock=c2838xlib/ADC
  Constant2 : Constant  Value=500e-3  OutDataTypeStr=fixdt(1,32,17)  SampleTime=-1
  Constant3 : Constant  Value=0.01  OutDataTypeStr=fixdt(1,32,17)  SampleTime=-1
  Divide : Product  Inputs=*/  OutDataTypeStr=fixdt(1,32,17)
  Gain : Gain  Gain=3.3/4095  OutDataTypeStr=fixdt(1,32,17)
  Subtract1 : Sum  Inputs=+-  OutDataTypeStr=fixdt(1,32,17)
  TCP_temp_Term1 : Terminator
  temperatureMOS : Outport
  wires:
  ADC1/1 -> Gain/1
  Subtract1/1 -> Divide/1
  Constant2/1 -> Subtract1/2
  Divide/1 -> temperatureMOS/1, TCP_temp_Term1/1
  Gain/1 -> Subtract1/1
  Constant3/1 -> Divide/2

== system focLib/Input Controller/speedMode_CodeGen ==
  Data Type Conversion : DataTypeConversion  OutDataTypeStr=fixdt(1,32,17)  SaturateOnIntegerOverflow=off  RndMeth=Floor
  Select first element : Selector  InputPortWidth=4  IndexOptions=Index vector (dialog)  Indices=[1]  OutputSizes=1
  Terminator : Terminator
  eCAN Receive1 : c280xlib/eCAN Receive  chipFamily=C280x  useModule=eCAN_A  mailboxNo=15  messageID=hex2dec('102')  messageType=Standard (11-bit identifier)  enableAcceptanceFiltering=off  messageIDMask=0  sampleTime=0.2  dataType=uint16  outputAction=Output last received values  initValue=0  outputMessageID=off  outputMessageLength=off  outputMessageTimeStamp=off  postInterrupt=off  interruptLine=0
      settings: LibrarySourceBlock=c28004xlib/eCAN Receive
  limit modes between 1 and 'availableSpeedModes' : Saturate  UpperLimit=availableSpeedModes  LowerLimit=1
  speedMode_CodeGen : Outport
  wires:
  limit modes between 1 and 'availableSpeedModes'/1 -> speedMode_CodeGen/1
  Data Type Conversion/1 -> limit modes between 1 and 'availableSpeedModes'/1
  Select first element/1 -> Data Type Conversion/1
  eCAN Receive1/1 -> Terminator/1
  eCAN Receive1/2 -> Select first element/1

== system focLib/Inverter and Motor - Plant Model/Codegeneration ==
  Duty_Cycles : Inport
  Ground : Ground
  Ground1 : Ground
  Terminator : Terminator
  Iab_fb_Sim : Outport  VectorParamsAs1DForOutWhenUnconnected=off
  Pos_fb_Sim : Outport  Port=2  VectorParamsAs1DForOutWhenUnconnected=off
  wires:
  Ground1/1 -> Pos_fb_Sim/1
  Ground/1 -> Iab_fb_Sim/1
  Duty_Cycles/1 -> Terminator/1

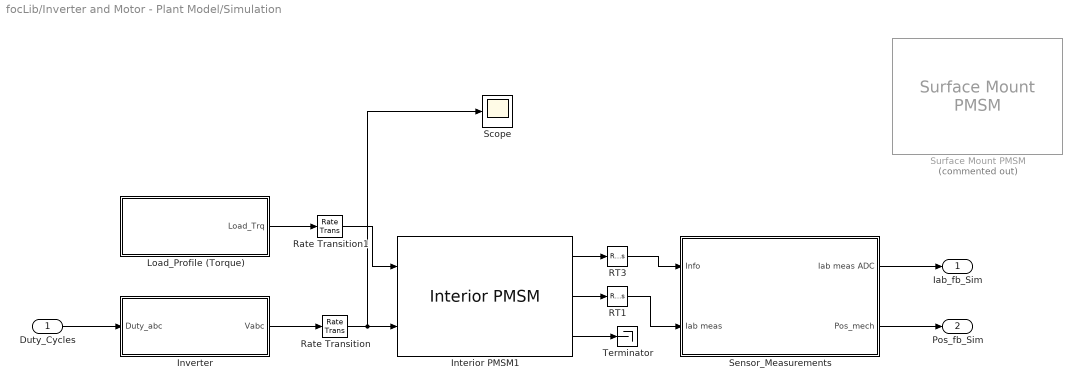
== system focLib/Inverter and Motor - Plant Model/Simulation ==
  Duty_Cycles : Inport
  Interior PMSM1 : autolibpmsminterior/Interior PMSM  port_config=Torque  sim_type=Discrete  Ts=Ts_motor  P=pmsm_ECI6360.p  Rs=pmsm_ECI6360.Rs  Ldq=[pmsm_ECI6360.Ld, pmsm_ECI6360.Lq]  KConstText=Permanent flux linkage constant (lambda_pm):  lambda_pm=pmsm_ECI6360.FluxPM  Ke=pmsm_ECI6360.Ke  mechanical=[pmsm_ECI6360.J,0,0]  idq0=[0 0]  theta_init=0  omega_init=0  KConst=pmsm_ECI6360.FluxPM  lambda_pm_calc=pmsm_ECI6360.FluxPM  Kt=0.07  RefBlkName='autolibpmsminterior/Interior PMSM'  aMode=5
      settings: LibrarySourceBlock=mcblib/Electrical Systems/Motors/Interior PMSM
  Inverter : Subsystem
  Load_Profile (Torque) : Subsystem
  RT1 : RateTransition  Deterministic=off  OutPortSampleTime=Ts_simulink
  RT3 : RateTransition  Deterministic=off  OutPortSampleTime=Ts_simulink
  Rate Transition : RateTransition  Deterministic=off  OutPortSampleTime=Ts_motor
  Rate Transition1 : RateTransition  Deterministic=off  OutPortSampleTime=Ts_motor
  Scope : Scope
  Sensor_Measurements : Subsystem
  Surface Mount PMSM : autolibpmsmexterior/Surface Mount PMSM  Commented=on  port_config=Torque  sim_type=Discrete  Ts=Ts_motor  P=4  Rs=1  Ldq_=pmsm_ECI6360.Ld  KConstText=Permanent flux linkage constant (lambda_pm):  lambda_pm=0.039  Ke=pmsm_ECI6360.Ke  Kt=1.323  mechanical=[pmsm_ECI6360.J, pmsm_ECI6360.B, 0]  idq0=[0 0]  theta_init=0  omega_init=0  KConst=0.039  lambda_pm_calc=0.039  RefBlkName='autolibpmsmexterior/Surface Mount PMSM'  aMode=5  Ldq="[0.0002      0.0002]"
  Terminator : Terminator
  Iab_fb_Sim : Outport  VectorParamsAs1DForOutWhenUnconnected=off
  Pos_fb_Sim : Outport  Port=2  VectorParamsAs1DForOutWhenUnconnected=off
  wires:
  Inverter/1(Vabc) -> Rate Transition/1
  Duty_Cycles/1 -> Inverter/1(Duty_abc)
  Rate Transition/1 -> Interior PMSM1/2, Scope/1
  Interior PMSM1/3 -> Terminator/1
  Interior PMSM1/2 -> RT1/1
  Interior PMSM1/1 -> RT3/1
  Load_Profile (Torque)/1(Load_Trq) -> Rate Transition1/1
  RT1/1 -> Sensor_Measurements/2(Iab meas)
  Rate Transition1/1 -> Interior PMSM1/1
  RT3/1 -> Sensor_Measurements/1(Info)
  Sensor_Measurements/2(Pos_mech) -> Pos_fb_Sim/1
  Sensor_Measurements/1(Iab meas ADC) -> Iab_fb_Sim/1

== system focLib/Speed Control/Digital_Freemode_Check ==
  Undervoltage_Sig : Inport
  Freemode : Inport  Port=2
  hot_temp : Inport  Port=3
  Check if Freemode is enabled : simulink/Logic and Bit Operations/Compare To Constant  relop===  const=1  OutDataTypeStr=boolean
  Check if MOSFETs are too hot : simulink/Logic and Bit Operations/Compare To Constant  relop===  const=1  OutDataTypeStr=boolean
  Check if Undervoltage is achieved : simulink/Logic and Bit Operations/Compare To Constant  relop===  const=1  OutDataTypeStr=boolean
  OR : Logic  Operator=OR  Inputs=3  AllPortsSameDT=off  OutDataTypeStr=boolean
  "Freemode_Sig  " : Outport
  wires:
  OR/1 -> "Freemode_Sig  "/1
  Check if MOSFETs are too hot/1 -> OR/3
  hot_temp/1 -> Check if MOSFETs are too hot/1
  Check if Freemode is enabled/1 -> OR/2
  Check if Undervoltage is achieved/1 -> OR/1
  Undervoltage_Sig/1 -> Check if Undervoltage is achieved/1
  Freemode/1 -> Check if Freemode is enabled/1

== system focLib/Speed Control/Mechanical_Freemode_Check ==
  Freemode_Sig_Dig : Inport
  SafeState : Inport  Port=2
  If : If  IfExpression=u1 ~= 1
  If Action Subsystem : Subsystem  TreatAsAtomicUnit=on
  If Action Subsystem1 : Subsystem  TreatAsAtomicUnit=on
  Merge : Merge
  Freemode_Sig : Outport
  wires:
  If/2 -> If Action Subsystem1/Action
  If Action Subsystem1/1(Out1) -> Merge/2
  If/1 -> If Action Subsystem/Action
  If Action Subsystem/1(Out1) -> Merge/1
  Freemode_Sig_Dig/1 -> If Action Subsystem1/1(Freemode_Sig_Dig)
  Merge/1 -> Freemode_Sig/1
  SafeState/1 -> If/1

== system focLib/Speed Control/PI_Controller_Speed ==
  N_ref : Inport
  N_fb : Inport  Port=2
  "  FreemodeEnabled?" : Inport  Port=3
  "Essential, so error of PI controller isn't rising" : Switch  Criteria=u2 > Threshold  OutDataTypeStr=fixdt(1,32,17)  SaturateOnIntegerOverflow=off  InputSameDT=off
  N_ref_abs : Abs  SaturateOnIntegerOverflow=off
  N_ref_small : simulink/Logic and Bit Operations/Compare To Constant  relop=<  const=ctrl_limits.N_ref_min  OutDataTypeStr=boolean
  PID Controller : slpidlib/PID Controller  Controller=PI  Form=Parallel  TimeDomain=Discrete-time  UseExternalTs=off  SampleTime=-1  IntegratorMethod=Forward Euler  FilterMethod=Forward Euler  ControllerParametersSource=internal  P=focp_tune_spd_Kp  I=focp_tune_spd_Ki  UseKiTs=off  D=0  N=100  UseFilter=on  TunerSelectOption=Transfer Function Based (PID Tuner App)  InitialConditionSource=internal  InitialConditionForIntegrator=0  InitialConditionForFilter=0  DifferentiatorICPrevScaledInput=0  ExternalReset=level  TrackingMode=off  Kt=1  LimitOutput=on  SatLimitsSource=internal  UpperSaturationLimit=focp_tune_iq_max  LowerSaturationLimit=focp_tune_iq_min  LinearizeAsGain=on  AntiWindupMode=clamping  Kb=1  LimitIntegrator=off  UpperIntegratorSaturationLimit=inf  LowerIntegratorSaturationLimit=-inf  RndMeth=Nearest  POutMin=[]  POutMax=[]  IOutMin=[]  IOutMax=[]  DOutMin=[]  DOutMax=[]  NOutMin=[]  NOutMax=[]  SumOutMin=[]  SumOutMax=[]  SaturationOutMin=[]  SaturationOutMax=[]  PParamDataTypeStr=fixdt(1,32,24)  PParamMin=[]  PParamMax=[]  IParamDataTypeStr=fixdt(1,32,24)  IParamMin=[]  IParamMax=[]  DParamMin=[]  DParamMax=[]  NParamMin=[]  NParamMax=[]  KbParamMin=[]  KbParamMax=[]  KtParamMin=[]  KtParamMax=[]  KbOutMin=[]  KbOutMax=[]  KtOutMin=[]  KtOutMax=[]  IntegratorOutMin=[]  IntegratorOutMax=[]  FilterOutMin=[]  FilterOutMax=[]  SumI1OutMin=[]  SumI1OutMax=[]  SumI2OutMin=[]  SumI2OutMax=[]  SumI3OutMin=[]  SumI3OutMax=[]  SumI4OutMin=[]  SumI4OutMax=[]  SumDOutMin=[]  SumDOutMax=[]  DifferentiatorOutMin=[]  DifferentiatorOutMax=[]  FilterDiffOutCoefMin=[]  FilterDiffOutCoefMax=[]  ReciprocalOutMin=[]  ReciprocalOutMax=[]  SumDenOutMin=[]  SumDenOutMax=[]  SumNumOutMin=[]  SumNumOutMax=[]  DivideOutMin=[]  DivideOutMax=[]  UdiffTsProdOutMin=[]  UdiffTsProdOutMax=[]  NTsProdOutMin=[]  NTsProdOutMax=[]  UintegralTsProdOutMin=[]  UintegralTsProdOutMax=[]  UngainTsProdOutMin=[]  UngainTsProdOutMax=[]  ClampingZeroOutDataTypeStr=Inherit: Inherit via back propagation  ClampingZeroOutMin=[]  ClampingZeroOutMax=[]  FilterDenConstantOutDataTypeStr=Inherit: Inherit via back propagation  FilterDenConstantOutMin=[]  FilterDenConstantOutMax=[]  PCopyOutDataTypeStr=Inherit: Inherit via back propagation  PCopyOutMin=[]  PCopyOutMax=[]  NCopyOutDataTypeStr=Inherit: Inherit via back propagation  NCopyOutMin=[]  NCopyOutMax=[]  IntegratorContinuousStateAttributes=''  IntegratorStateMustResolveToSignalObject=off  IntegratorRTWStateStorageClass=Auto  FilterContinuousStateAttributes=''  FilterStateMustResolveToSignalObject=off  FilterRTWStateStorageClass=Auto  ParallelPVariant=InternalParameters  IdealPVariant=Disabled  IVariant=InternalParameters  DVariant=Disabled  IntegratorVariant=Discrete  SatVariant=Enabled  AWVariant=DiscClampingParallel  PCopyVariant=Disabled  TRVariant=Disabled  FdbkBlocksVariant=Forward  IdealPFdbkVariant=Disabled  SatFdbkVariant=Disabled  DerivativeFilterVariant=Disabled  NVariant=Disabled  NCopyVariant=Disabled_SignalSpec  FilterICVariant=Disabled  IntegratorICVariant=InternalICs  ExternalResetVariant=ExternalReset  TRSumVariant=Passthrough  SumFdbkVariant=Disabled  SumVariant=Sum_PI  TsampFilterVariant=InternalTs  TsampNgainVariant=Passthrough  TsampIntegralVariant=Disabled_SignalSpec  ExternalSaturationOutDataTypeStr=Inherit: Same as second input
  Reset_I_And : Logic  AllPortsSameDT=off  OutDataTypeStr=boolean
  Reset_I_Freemode_Enable : Constant  Value=ctrl_limits.reset_I_freemode  OutDataTypeStr=boolean
  Reset_I_Or : Logic  Operator=OR  AllPortsSameDT=off  OutDataTypeStr=boolean
  Saturation : Saturate  UpperLimit=0  LowerLimit=0
  Sum : Sum  Inputs=|+-  RndMeth=Round
  Iq_ref : Outport  VectorParamsAs1DForOutWhenUnconnected=off
  wires:
  "Essential, so error of PI controller isn't rising"/1 -> Sum/1
  Sum/1 -> PID Controller/1
  Saturation/1 -> "Essential, so error of PI controller isn't rising"/1
  "  FreemodeEnabled?"/1 -> "Essential, so error of PI controller isn't rising"/2, Reset_I_And/1
  PID Controller/1 -> Iq_ref/1
  N_fb/1 -> Sum/2
  N_ref/1 -> "Essential, so error of PI controller isn't rising"/3, Saturation/1, N_ref_abs/1
  Reset_I_Freemode_Enable/1 -> Reset_I_And/2
  N_ref_abs/1 -> N_ref_small/1
  Reset_I_And/1 -> Reset_I_Or/1
  N_ref_small/1 -> Reset_I_Or/2
  Reset_I_Or/1 -> PID Controller/2
